simulink model "DSD_control_system"  (R2023a)
settings: Solver=VariableStepAuto  StartTime=0.0  StopTime=30  RelTol=1e-3
settings Model: DataDictionary=DSD_system_data.sldd  EnableAccessToBaseWorkspace=off  Creator=tshintai  LastModifiedBy=tshintai
settings SolverCC: AlgebraicLoopSolver=TrustRegion
settings OptimizationCC: ReuseModelBlockBuffer=off
settings DebuggingCC: UnconnectedInputMsg=warning  UnconnectedOutputMsg=warning  UnconnectedLineMsg=warning
settings ModelReferenceCC: EnableRefExpFcnMdlSchedulingChecks=on
settings RTWCC: DLArmComputeVersion=19.05

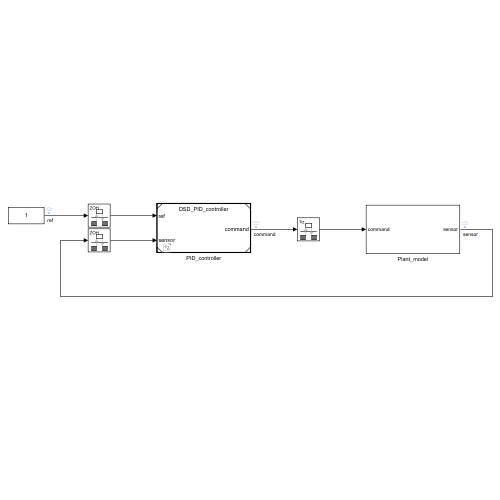
[thumbnail: Simulink's stored preview of the top-level diagram]
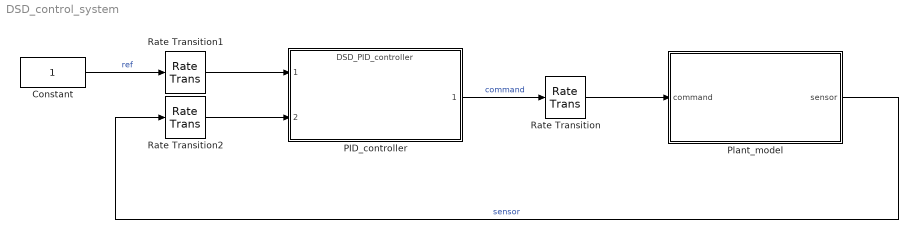
== system DSD_control_system ==
  Constant : Constant
  PID_controller : ModelReference  ModelNameDialog=DSD_PID_controller  SimulationMode=Normal  ModelReferenceVersion=6.0
  Plant_model : Subsystem
  Rate Transition : RateTransition
  Rate Transition1 : RateTransition  OutPortSampleTime=ts
  Rate Transition2 : RateTransition  OutPortSampleTime=ts
  wires:
  Constant/1 -> Rate Transition1/1  "ref"
  PID_controller/1 -> Rate Transition/1  "command"
  Plant_model/1(sensor) -> Rate Transition2/1  "sensor"
  Rate Transition/1 -> Plant_model/1(command)
  Rate Transition1/1 -> PID_controller/1
  Rate Transition2/1 -> PID_controller/2

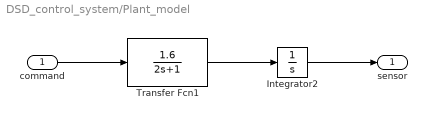
== system DSD_control_system/Plant_model ==
  command : Inport
  Integrator2 : Integrator
  Transfer Fcn1 : TransferFcn  Numerator=[1.6]  Denominator=[2 1]
  sensor : Outport
  wires:
  Transfer Fcn1/1 -> Integrator2/1
  Integrator2/1 -> sensor/1
  command/1 -> Transfer Fcn1/1
